simulink model "A_ZH_Z2"  (R2026a)
settings: Solver=VariableStepAuto  StopTime=10
settings Model: Creator=Szalay  LastModifiedBy=Szalay

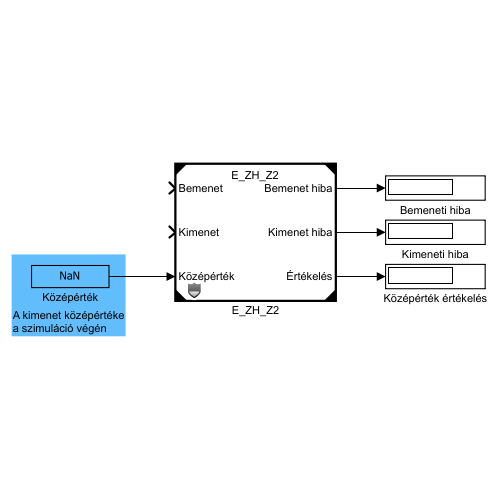
[thumbnail: Simulink's stored preview of the top-level diagram]
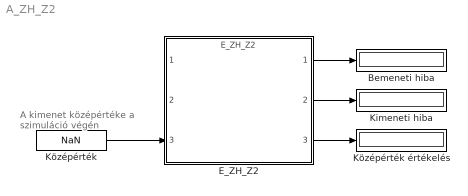
== system A_ZH_Z2 ==
  note: A kimenet középértéke
      | a szimuláció végén
  Bemeneti hiba : Display
  E_ZH_Z2 : ModelReference  ModelNameDialog=E_ZH_Z2.slxp  ModelReferenceVersion=3.0  CopyOfModelProtected=on
  Kimeneti hiba : Display
  Középérték : Constant  Value=NaN
  Középérték értékelés : Display
  wires:
  E_ZH_Z2/1 -> Bemeneti hiba/1
  E_ZH_Z2/2 -> Kimeneti hiba/1
  E_ZH_Z2/3 -> Középérték értékelés/1
  Középérték/1 -> E_ZH_Z2/3
